simulink model "observer_simple"  (R2025b)
settings: Solver=ode45  StartTime=0.0  StopTime=8  MaxStep=0.01  RelTol=1e-8  AbsTol=1e-10
settings Model: Creator=alosw  LastModifiedBy=alosw

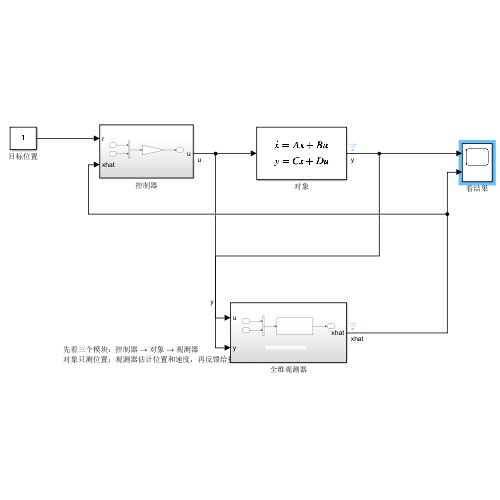
[thumbnail: Simulink's stored preview of the top-level diagram]
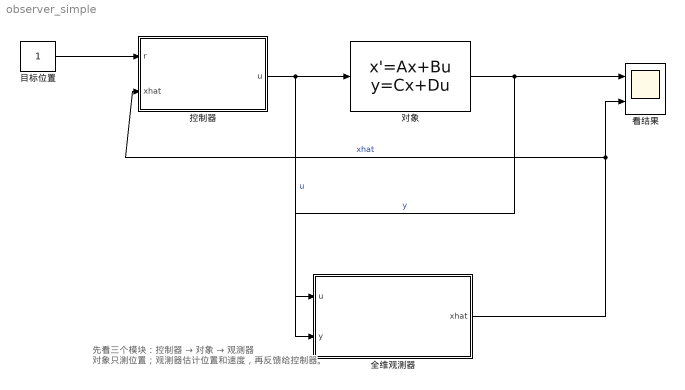
== system observer_simple ==
  note: 先看三个模块：控制器 → 对象 → 观测器
      | 对象只测位置；观测器估计位置和速度，再反馈给控制器。
  全维观测器 : Subsystem
  对象 : StateSpace  A=[0 1;-2 -3]  B=[0;1]  C=[1 0]  D=0  InitialCondition=[0.5;0]
  控制器 : Subsystem
  目标位置 : Constant
  看结果 : Scope  NumInputPorts=2
      settings: ActiveDisplayYMinimum=0.22952726724103883  ActiveDisplayYMaximum=0.99691867590093164
  wires:
  目标位置/1 -> 控制器/1(r)
  控制器/1(u) -> 对象/1, 全维观测器/1(u)  "u"
  对象/1 -> 全维观测器/2(y), 看结果/1  "y"
  全维观测器/1(xhat) -> 看结果/2, 控制器/2(xhat)  "xhat"

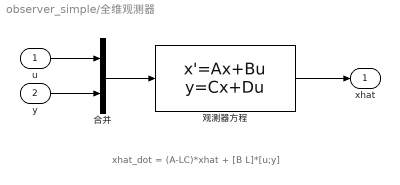
== system observer_simple/全维观测器 ==
  note: xhat_dot = (A-LC)*xhat + [B L]*[u;y]
  u : Inport
  y : Inport  Port=2
  合并 : Mux  Inputs=2
  观测器方程 : StateSpace  A=[-8 1;-6 -3]  B=[0 8;1 4]  C=eye(2)  D=zeros(2,2)  InitialCondition=[0;0]
  xhat : Outport
  wires:
  u/1 -> 合并/1
  y/1 -> 合并/2
  合并/1 -> 观测器方程/1
  观测器方程/1 -> xhat/1

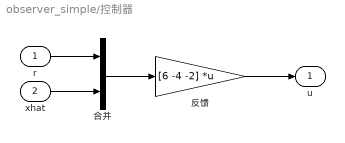
== system observer_simple/控制器 ==
  r : Inport
  xhat : Inport  Port=2
  反馈 : Gain  Gain=[6 -4 -2]  Multiplication=Matrix(K*u)
  合并 : Mux  Inputs=2
  u : Outport
  wires:
  r/1 -> 合并/1
  xhat/1 -> 合并/2
  合并/1 -> 反馈/1
  反馈/1 -> u/1
